simulink model "reference_05_two_coupled_loops"  (R2026b)
settings: Solver=FixedStepDiscrete  StartTime=0  StopTime=0.5  FixedStep=0.01  RelTol=1e-10  AbsTol=1e-12
settings Model: Creator=Fasih  LastModifiedBy=Fasih
settings DataIOCC: SaveOutput=off

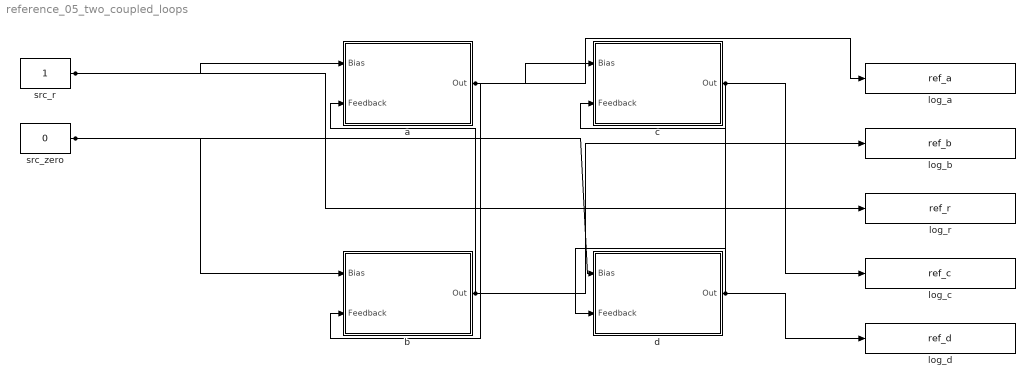
== system reference_05_two_coupled_loops ==
  a : Subsystem
  b : Subsystem
  c : Subsystem
  d : Subsystem
  log_a : ToWorkspace  VariableName=ref_a  SaveFormat=Timeseries  SampleTime=0.01
  log_b : ToWorkspace  VariableName=ref_b  SaveFormat=Timeseries  SampleTime=0.01
  log_c : ToWorkspace  VariableName=ref_c  SaveFormat=Timeseries  SampleTime=0.01
  log_d : ToWorkspace  VariableName=ref_d  SaveFormat=Timeseries  SampleTime=0.01
  log_r : ToWorkspace  VariableName=ref_r  SaveFormat=Timeseries  SampleTime=0.01
  src_r : Constant  OutDataTypeStr=double
  src_zero : Constant  Value=0  OutDataTypeStr=double
  wires:
  src_r/1 -> a/1(Bias), log_r/1
  src_zero/1 -> b/1(Bias), d/1(Bias)
  b/1(Out) -> a/2(Feedback), log_b/1
  a/1(Out) -> b/2(Feedback), log_a/1, c/1(Bias)
  c/1(Out) -> d/2(Feedback), log_c/1
  d/1(Out) -> c/2(Feedback), log_d/1

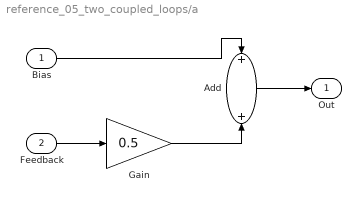
== system reference_05_two_coupled_loops/a ==
  Bias : Inport
  Feedback : Inport  Port=2
  Add : Sum
  Gain : Gain  Gain=0.5
  Out : Outport
  wires:
  Bias/1 -> Add/1
  Feedback/1 -> Gain/1
  Gain/1 -> Add/2
  Add/1 -> Out/1

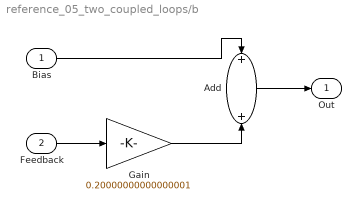
== system reference_05_two_coupled_loops/b ==
  Bias : Inport
  Feedback : Inport  Port=2
  Add : Sum
  Gain : Gain  Gain=0.20000000000000001
  Out : Outport
  wires:
  Bias/1 -> Add/1
  Feedback/1 -> Gain/1
  Gain/1 -> Add/2
  Add/1 -> Out/1

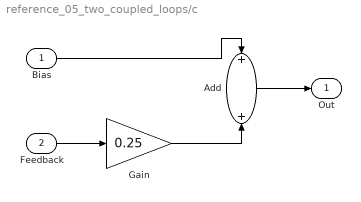
== system reference_05_two_coupled_loops/c ==
  Bias : Inport
  Feedback : Inport  Port=2
  Add : Sum
  Gain : Gain  Gain=0.25
  Out : Outport
  wires:
  Bias/1 -> Add/1
  Feedback/1 -> Gain/1
  Gain/1 -> Add/2
  Add/1 -> Out/1

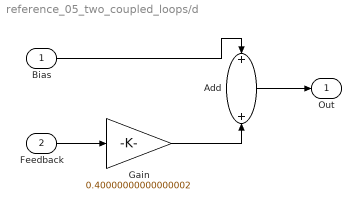
== system reference_05_two_coupled_loops/d ==
  Bias : Inport
  Feedback : Inport  Port=2
  Add : Sum
  Gain : Gain  Gain=0.40000000000000002
  Out : Outport
  wires:
  Bias/1 -> Add/1
  Feedback/1 -> Gain/1
  Gain/1 -> Add/2
  Add/1 -> Out/1
